simulink model "Single_phase_fully_controlled_bridge_converter_fed_separately_excited_DC_motor"  (R2024a)
settings: Solver=VariableStepAuto  StartTime=0.0  StopTime=5  RelTol=1e-3
libraries: spsThyristorLib x4, spsACVoltageSourceLib x1, spsCurrentMeasurementLib x1, spsDCMachineLib x1, spsDCVoltageSourceLib x1, simulink x1, spsVoltageMeasurementLib x1, sps_lib x1
settings Model: Creator=haris  LastModifiedBy=haris

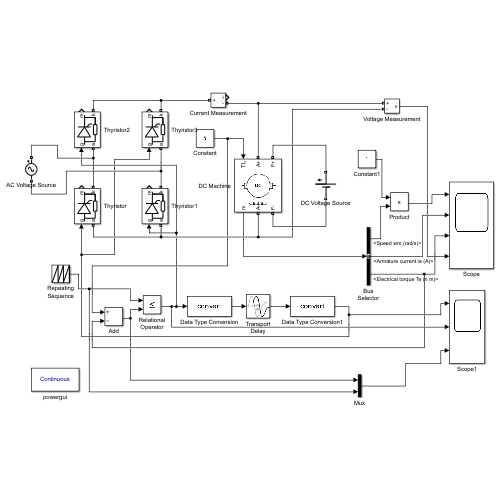
[thumbnail: Simulink's stored preview of the top-level diagram]
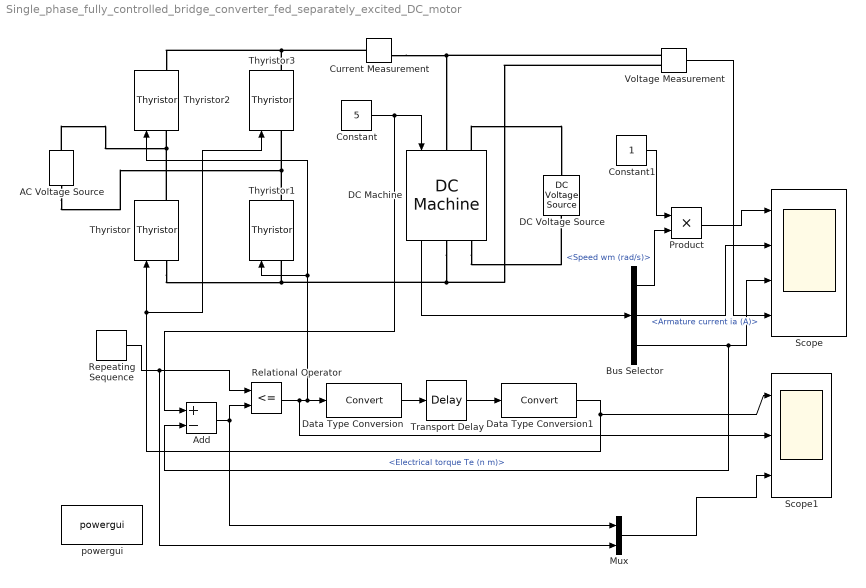
== system Single_phase_fully_controlled_bridge_converter_fed_separately_excited_DC_motor ==
  AC Voltage Source : spsACVoltageSourceLib/AC Voltage Source  Amplitude=325  Phase=0  Frequency=50  SampleTime=0  Measurements=None  BusType=swing  Pref=10e3  Qref=0  Qmin=-inf  Qmax=+inf
  Add : Sum  Inputs=+-
  Bus Selector : BusSelector  OutputSignals=Speed wm (rad/s),Armature current ia (A),Electrical torque Te (n m)
  Constant : Constant  Value=5
  Constant1 : Constant
  Current Measurement : spsCurrentMeasurementLib/Current Measurement  PhasorSimulation=off  OutputType=Complex  PSBequivalent=0
  DC Machine : spsDCMachineLib/DC Machine  PresetModel=No  MechanicalLoad=Torque TL  FieldType=Wound  ShowDetailedParameters=on  MeasurementBus=off  RLa="[ 0.6  0.012]"  RLf="[ 240  120]"  Laf=1.8  MachineConstant=Torque constant (N.m/A)  Ke=1.8  Kt=1.8  J=1  Bm=0  Tf=0  w0=1  Ifinit=1.2499999987663  TsPowergui=0  TsBlock=-1
  DC Voltage Source : spsDCVoltageSourceLib/DC Voltage Source  Amplitude=300  Measurements=None
  Data Type Conversion : DataTypeConversion  SaturateOnIntegerOverflow=off  RndMeth=Floor
  Data Type Conversion1 : DataTypeConversion  SaturateOnIntegerOverflow=off  RndMeth=Floor
  Mux : Mux  Inputs=2
  Product : Product
  Relational Operator : RelationalOperator  Operator=<=  OutDataTypeStr=boolean  RndMeth=Simplest  InputSameDT=off
  Repeating Sequence : simulink/Sources/Repeating Sequence  rep_seq_t=[0 2]  rep_seq_y=[0 2]
  Scope : Scope  NumInputPorts=4
  Scope1 : Scope  NumInputPorts=3
  Thyristor{,1..3} (4 alike) : spsThyristorLib/Thyristor  Ron=0.001  Lon=0  Vf=0.8  IC=0  Rs=500  Cs=250e-9  Measurements=on
  Transport Delay : TransportDelay  DelayTime=0.01
  Voltage Measurement : spsVoltageMeasurementLib/Voltage Measurement  PhasorSimulation=off  OutputType=Complex  PSBequivalent=0
  powergui : sps_lib/powergui  Priority=1  SimulationMode=Continuous  SampleTime=50e-6  frequency=60  Iterations=50  frequencyindice=50  Pbase=100e6  ErrMax=1e-4  UnitsV=kV  UnitsW=MW  buscounter=0  FunctionMessages=off  echomessages=off  EnableUseOfTLC=off  CurrentSourceSwitches=off  DisableSnubberDevices=off  DisableRonSwitches=off  DisableVfSwitches=off  DisplayEquations=off  AutomaticDiscreteSolvers=off  SolverType=Tustin/Backward Euler (TBE)  Interpol=off  ExternalGateDelay=off  methode=off  Ts=100  x0status=blocks  SPID=on  SwTol=0  HookPort=off  NonlinearTolerance=1e-4  nMaxIteration=100  ContinueOnMaxIteration=off  RestoreLinks=warning  ResistiveCurrentMeasurement=off  Frange=[0:2:500]  Ylog=off  Xlog=on  ShowGrid=off  save=off  variable=ZData  structure=0  ZoomFFT=off  StartTime=0.0  cycles=1  DisplayStyle=1  fundamental=60  FreqAxis=off  MaxFrequency=1000  frequencyindicesteady=1  RmsSteady=1  display=off
  wires:
  Constant/1 -> Add/1, DC Machine/1
  DC Machine/1 -> Bus Selector/1
  Constant1/1 -> Product/1
  Bus Selector/1 -> Product/2  "<Speed wm (rad/s)>"
  Product/1 -> Scope/1
  Bus Selector/2 -> Scope/2  "<Armature current ia (A)>"
  Bus Selector/3 -> Add/2, Scope/3  "<Electrical torque Te (n m)>"
  Voltage Measurement/1 -> Scope/4
  Repeating Sequence/1 -> Relational Operator/1, Mux/2
  Add/1 -> Mux/1, Relational Operator/2
  Relational Operator/1 -> Scope1/2, Thyristor1/1, Thyristor2/1, Data Type Conversion/1
  Data Type Conversion/1 -> Transport Delay/1
  Transport Delay/1 -> Data Type Conversion1/1
  Data Type Conversion1/1 -> Thyristor3/1, Thyristor/1, Scope1/1
  Mux/1 -> Scope1/3
  connections:
  Thyristor/RConn1 -- AC Voltage Source/RConn1 -- Thyristor2/LConn1
  Thyristor1/RConn1 -- AC Voltage Source/LConn1 -- Thyristor3/LConn1
  Thyristor3/RConn1 -- Current Measurement/LConn1 -- Thyristor2/RConn1
  Current Measurement/RConn1 -- Voltage Measurement/LConn1 -- DC Machine/LConn1
  Thyristor/LConn1 -- Voltage Measurement/LConn2 -- DC Machine/RConn1 -- Thyristor1/LConn1
  DC Machine/LConn2 -- DC Voltage Source/RConn1
  DC Machine/RConn2 -- DC Voltage Source/LConn1
